simulink model "Simulation_cs"  (R2019a)
settings: Solver=ode5  StartTime=0.0  StopTime=inf  FixedStep=1/20  RelTol=1e-3
PreLoadFcn:
  | mbxruntime.callbacks.PreLoadFcn(bdroot);
PostLoadFcn:
  | mbxruntime.callbacks.PostLoadFcn(bdroot);
InitFcn:
  | mbxruntime.callbacks.InitFcn(bdroot);
StartFcn:
  | mbxruntime.callbacks.StartFcn(bdroot);
StopFcn:
  | mbxruntime.callbacks.StopFcn(bdroot);
model workspace: external: MAT-File .\Simulation_cs_hws.mat (data not in the file)
undefined symbols (not defined in the file or in its folder): DiscIntNeverNeededParam, InitImageOutputDir, mbxruntime, Simulation_cs_3ba1e87c6cdc7fd9, Simulation_cs_BMW_X5_SUV_1_Dynamics_Empty_STATE_BMW_X5_SUV_1_x0, Simulation_cs_BMW_X5_SUV_1_Dynamics_Empty_STATE_BMW_X5_SUV_1_y0, Simulation_cs_BMW_X5_SUV_1_Dynamics_Empty_STATE_BMW_X5_SUV_1_z0, Simulation_cs_dbe7801ee2d75073, Simulation_cs_f34d2d8469e03015
libraries: adeye_lib x45, robotlib x3, PreScanSimulinkLibrary x2, PreScanUsefulBlocks x1
(part 1 of 3)
CloseFcn:
  | mbxruntime.callbacks.CloseFcn(bdroot);
settings Model: Creator=PRESCAN  LastModifiedBy=adeye05w
settings DataIOCC: LimitDataPoints=on  SaveFormat=Array  SignalLoggingSaveFormat=ModelDataLogs  ReturnWorkspaceOutputs=off
settings OptimizationCC: DefaultParameterBehavior=Inlined  ExpressionDepthLimit=2147483647  InitFltsAndDblsToZero=on  LifeSpan=inf
settings DebuggingCC: SaveWithParameterizedLinksMsg=none  UnderspecifiedInitializationDetection=Classic  MergeDetectMultiDrivingBlocksExec=none  SignalResolutionControl=TryResolveAllWithWarning  MultiTaskDSMMsg=warning  MultiTaskCondExecSysMsg=none  FcnCallInpInsideContextMsg=warning  StateNameClashWarn=warning  SFUnexpectedBacktrackingDiag=warning  SFNoUnconditionalDefaultTransitionDiag=warning  SFExecutionAtInitializationDiag=none  ArithmeticOperatorsInVariantConditions=warning
settings HardwareCC: ProdBitPerPointer=32  ProdBitPerSizeT=32  ProdBitPerPtrDiffT=32  ProdLargestAtomicFloat=None  ProdIntDivRoundTo=Undefined  ProdEndianess=Unspecified  ProdWordSize=32  ProdHWDeviceType=32-bit Generic
settings ModelReferenceCC: UpdateModelReferenceTargets=IfOutOfDate  PropagateSignalLabelsOutOfModel=off
settings SFSimCC: SimUseLocalCustomCode=off  SimParseCustomCode=off
settings SFSimCC: SimCustomHeaderCode=|
  | #include "prescan.h"
  | #include "prescan_platform.h"
  | #include "prescan_aimsunturnindicatorsetter_data.h"
settings RTWCC: RTWUseLocalCustomCode=off
settings CodeAppCC: StateflowObjectComments=on
settings GRTTargetCC: TargetFcnLib=ansi_tfl_tmw.mat  TargetLangStandard=C89/C90 (ANSI)  GeneratePreprocessorConditionals=Disable all  CombineOutputUpdateFcns=off  GRTInterface=on
settings ConfigComp: CovMetricSettings=dw  CovHtmlReporting=on  CovSaveCumulativeToWorkspaceVar=on  CovSaveSingleToWorkspaceVar=on  CovExternalEMLEnable=off  CovSFcnEnable=off

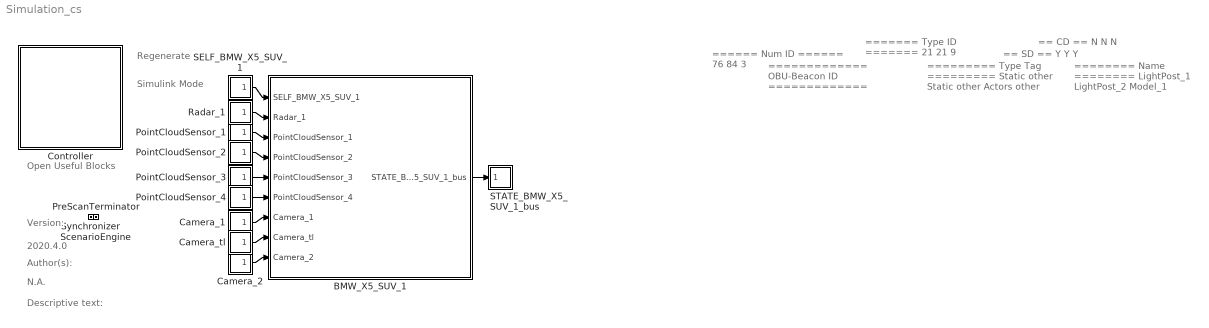
== system Simulation_cs ==
  note: Regenerate
  note: Simulink Mode
  note: Open Useful Blocks
  note: 2020.4.0
  note: Version:
  note: Author(s):
  note: N.A.
  note: Descriptive text:
  note: ======
      | Num ID
      | ======
      | 76
      | 84
      | 3
  note: =============
      | OBU-Beacon ID
      | =============
  note: =======
      | Type ID
      | =======
      | 21
      | 21
      | 9
  note: =========
      | Type Tag
      | =========
      | Static other
      | Static other
      | Actors other
  note: ==
      | SD
      | ==
      | Y
      | Y
      | Y
  note: ==
      | CD
      | ==
      | N
      | N
      | N
  note: ========
      | Name
      | ========
      | LightPost_1
      | LightPost_2
      | Model_1
  BMW_X5_SUV_1 : Subsystem  Tag=WorldObjectSubSystem  InitFcn=UniqueId = '158';
      mask init:
      | modelPath = GenericModelHelper.getGenericModelFilePath('ModelDepo','Vehicles\BMW_X5\BMW_X5.pgmb','bfeb1c11467705ab888b3011684c848b');imagePath = GenericModelHelper.getCompilationPicture(modelPath, 'BMW_X5_HighPoly.png');
      mask Display: image(imread(imagePath));color('white');text(0, 0, ' ID=10\n')
  Camera_1 : Subsystem  Tag=sensor/Camera/CameraSensor  Priority=30  mask(PreScan Source Block: Camera Sensor){}
      mask help: The Camera Sensor provides a color or monochrome image.
      settings: OpenFcn=open_system([gcb '/Sensor'],'mask')
      mask Help: eval('openHelp(457)')
      mask Display: image(imread('CameraSensor.png'))
  Camera_2 : Subsystem  Tag=sensor/Camera/CameraSensor  Priority=30  mask(PreScan Source Block: Camera Sensor){}
      mask help: The Camera Sensor provides a color or monochrome image.
      settings: OpenFcn=open_system([gcb '/Sensor'],'mask')
      mask Help: eval('openHelp(457)')
      mask Display: image(imread('CameraSensor.png'))
  Camera_tl : Subsystem  Tag=sensor/Camera/CameraSensor  Priority=30  mask(PreScan Source Block: Camera Sensor){}
      mask help: The Camera Sensor provides a color or monochrome image.
      settings: OpenFcn=open_system([gcb '/Sensor'],'mask')
      mask Help: eval('openHelp(457)')
      mask Display: image(imread('CameraSensor.png'))
  Controller : Subsystem  Description=8A3CD2955739A82C886C20AE3E253D78460D53180EE2C1B14CC08DF75A70BE77  Priority=-1  LoadFcn=load PreScanControllerData  mask(PreScan Simulation Controller){prescanversion='2020.4.0', ModelReferencing=off, TimeStep=1/20, ControlMode=0, PreScanExecutionMode=on, ControllerCount=0, ControllerIndex=0, ControllerOptions=''}
      mask prompts: prescanversion "PreScan Version"; ModelReferencing "Use Model Referencing"; TimeStep "Upload Period [s]"; ControlMode "Control Mode"; PreScanExecutionMode "Execution Mode"; ControllerCount "Controller Count"; ControllerIndex "Controller Index"; ControllerOptions "Controller Options"
      mask help:
      | Please do not remove this block from the compilation sheet,
      | as it connects the model to the PreScan environment.
      mask init:
      | model = bdroot(gcb);
      | ExperimentFile = mbxruntime.findExperimentFile(model,true); %relative path
      | 
      | [d1, d2, d3, prescandata] = prescan_Settings();
      | ModelDepo = fullfile(prescandata,'ModelDepo'); 
      | 
      | RTmode = mbxruntime.getRTMode(model);
      | 
      | SimulationMode = get_param(bdroot,'SimulationMode');
      | if strcmp(SimulationMode, 'rapid-accelerator')
      |     SimulationMode = 'external';
      | end
      | TargetName = get_param(bdroot,'SystemTargetFile');
      settings: ModelCloseFcn=assignin('base',['model_closed_' bdroot],true);
      mask Help: eval('openHelp(812)')
      mask Display: image(imread('prescanlogo.ico'))
  PointCloudSensor_1 : Subsystem  Tag=sensor/PointCloudInport  Priority=30  mask(PreScan Source Block: Point Cloud Sensor){}
      mask help: The Point Cloud Sensor provides XYZ positions relative to the sensor
      settings: OpenFcn=open_system([gcb '/Sensor'],'mask')
      mask Help: eval('openHelp(6400)')
      mask Display: image(imread('PointCloudSensorSL.png'))
  PointCloudSensor_2 : Subsystem  Tag=sensor/PointCloudInport  Priority=30  mask(PreScan Source Block: Point Cloud Sensor){}
      mask help: The Point Cloud Sensor provides XYZ positions relative to the sensor
      settings: OpenFcn=open_system([gcb '/Sensor'],'mask')
      mask Help: eval('openHelp(6400)')
      mask Display: image(imread('PointCloudSensorSL.png'))
  PointCloudSensor_3 : Subsystem  Tag=sensor/PointCloudInport  Priority=30  mask(PreScan Source Block: Point Cloud Sensor){}
      mask help: The Point Cloud Sensor provides XYZ positions relative to the sensor
      settings: OpenFcn=open_system([gcb '/Sensor'],'mask')
      mask Help: eval('openHelp(6400)')
      mask Display: image(imread('PointCloudSensorSL.png'))
  PointCloudSensor_4 : Subsystem  Tag=sensor/PointCloudInport  Priority=30  mask(PreScan Source Block: Point Cloud Sensor){}
      mask help: The Point Cloud Sensor provides XYZ positions relative to the sensor
      settings: OpenFcn=open_system([gcb '/Sensor'],'mask')
      mask Help: eval('openHelp(6400)')
      mask Display: image(imread('PointCloudSensorSL.png'))
  PreScanTerminator : Subsystem  Tag=PreScanTerminator  Priority=999  LoadFcn=load PrescanTerminatorData  mask(PreScan Simulation Terminator){TimeStep=1/20}
      mask prompts: TimeStep "Upload Period [s]"
      mask help:
      | Please do not remove this block from the compilation sheet as it
      | connects the model to the PreScan environment.
      mask Help: eval('openHelp(812)')
      mask Display: image(imread('prescanlogo.ico'))
  Radar_1 : Subsystem  Tag=sensor/Radar  Priority=30  LoadFcn=load('PrescanScannerSensorData.mat');load('PrescanScannerSensorMessage.mat')  mask(PreScan Source Block: Radar Sensor){}
      mask help:
      | The Radar Sensor is a detailed sensor based on a physical radar
      | model that includes Antenna GAIN Maps (AGM) and atmospheric
      | attenuation.
      |
      | For more information, please click Help.
      settings: OpenFcn=open_system([gcb '/Sensor'],'mask')
      mask Help: eval('openHelp(1464)')
      mask Display: image(imread('Radar.png'))
  SELF_BMW_X5_SUV_1 : Subsystem  Tag=sensor/SelfPort  Priority=30  LoadFcn=load('PreScanSelfSensorData.mat')  mask(PreScan Source Block: SELF){}
      mask help:
      | The SELF port shows (state) information of the actor itself. The outputs are position in the experiment's axis system and the GPS coordinates, and the object's absolute velocity and compass heading.
      |
      | For more information, please click Help.
      settings: OpenFcn=open_system([gcb '/Sensor'],'mask')
      mask Help: eval('openHelp(462)')
      mask Display: image(imread('GPS.png'))
  STATE_BMW_X5_SUV_1_bus : Subsystem  Tag=actuator/StatePort  Priority=0  LoadFcn=load('PreScanStateActuatorData.mat')  mask(PreScan Sink Block: State){}
      mask help:
      | The Actor State contains a vector signal of size (9x1), containing the following signals:
      |
      | -  Position    	(x,y,z)             	[m]
      | -  Velocity    	(vx,vy,vz)         	[m/s]
      | -  Angles       	(Roll, Pitch, Yaw)	[rad]
      |
      | The Actor state is defined in the global axis system.
      | The state is superponed on the Initial position defined in the GUI.
      |
      | For more information, please click Help.
      settings: OpenFcn=open_system([gcb '/Actuator'],'mask')
      mask Help: eval('openHelp(222)')
      mask Display: image(imread('State.png'))
  ScenarioEngine : Subsystem  Tag=PreScanOpenScenarioBlock  Priority=10  LoadFcn=load PrescanSynchronizeData  mask(PreScan Simulation Core Block){TimeStep=1/20}
      mask prompts: TimeStep "Timestep [s]"
      mask help:
      | Please do not remove this block from the PreScan compilation sheet,
      | as it contains essential configuration parameters for a PreScan simulation.
      settings: DeleteFcn=PreScanBlockDeleteFcn;
      mask Display: image(imread('prescanlogo.ico'))
  Synchronizer : Subsystem  Tag=PreScanSynchronizer  Priority=20  LoadFcn=load PrescanSynchronizeData  mask(PreScan Simulation Core Block){TimeStep=1/20}
      mask prompts: TimeStep "Timestep [s]"
      mask help:
      | Please do not remove this block from the PreScan compilation sheet,
      | as it contains essential configuration parameters for a PreScan simulation.
      settings: DeleteFcn=PreScanBlockDeleteFcn;
      mask Display: image(imread('prescanlogo.ico'))
  wires:
  BMW_X5_SUV_1/1(STATE_BMW_X5_SUV_1_bus) -> STATE_BMW_X5_SUV_1_bus/1(STATE_BMW_X5_SUV_1_bus)
  SELF_BMW_X5_SUV_1/1(SELF_BMW_X5_SUV_1) -> BMW_X5_SUV_1/1(SELF_BMW_X5_SUV_1)
  Radar_1/1(Radar_1) -> BMW_X5_SUV_1/2(Radar_1)
  PointCloudSensor_1/1(PointCloudSensor_1) -> BMW_X5_SUV_1/3(PointCloudSensor_1)
  PointCloudSensor_2/1(PointCloudSensor_2) -> BMW_X5_SUV_1/4(PointCloudSensor_2)
  PointCloudSensor_3/1(PointCloudSensor_3) -> BMW_X5_SUV_1/5(PointCloudSensor_3)
  PointCloudSensor_4/1(PointCloudSensor_4) -> BMW_X5_SUV_1/6(PointCloudSensor_4)
  Camera_1/1(Camera_1) -> BMW_X5_SUV_1/7(Camera_1)
  Camera_tl/1(Camera_tl) -> BMW_X5_SUV_1/8(Camera_tl)
  Camera_2/1(Camera_2) -> BMW_X5_SUV_1/9(Camera_2)
